simulink subsystem "Vision_Corrections_sub"  (R2023b)
settings: Solver=VariableStepAuto  StartTime=0.0  StopTime=10.0  RelTol=1e-3
undefined symbols (not defined in the file): Vision_Object_Angle_Offset, Vision_Object_X_Offset, Vision_Object_Y_Offset, Vision_Tag_Angle_Offset, Vision_Tag_X_Offset, Vision_Tag_Y_Offset
libraries: simulink_extras x2
settings Model: Creator=ander  LastModifiedBy=ander

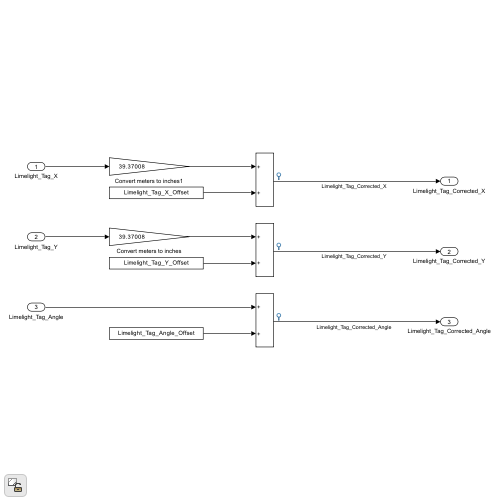
[thumbnail: Simulink's stored preview of the top-level diagram]
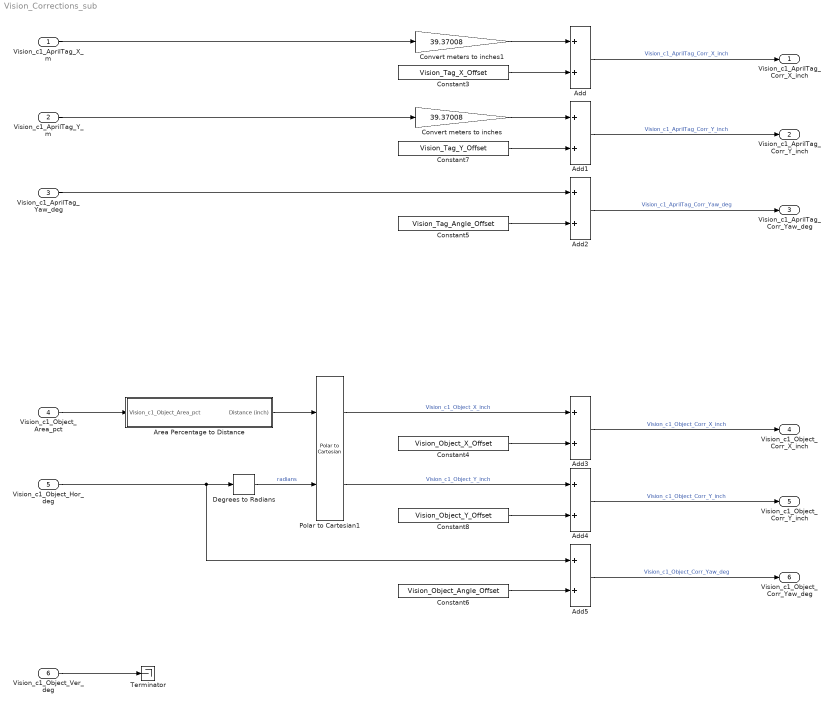
== system Vision_Corrections_sub ==
  Vision_c1_AprilTag_X_m : Inport
  Vision_c1_AprilTag_Y_m : Inport  Port=2
  Vision_c1_AprilTag_Yaw_deg : Inport  Port=3
  Vision_c1_Object_Area_pct : Inport  Port=4
  Vision_c1_Object_Hor_deg : Inport  Port=5
  Vision_c1_Object_Ver_deg : Inport  Port=6
  Add{,1..5} (6 alike) : Sum
  Area Percentage to Distance : Subsystem
  Constant3 : Constant  Value=Vision_Tag_X_Offset
  Constant4 : Constant  Value=Vision_Object_X_Offset
  Constant5 : Constant  Value=Vision_Tag_Angle_Offset
  Constant6 : Constant  Value=Vision_Object_Angle_Offset
  Constant7 : Constant  Value=Vision_Tag_Y_Offset
  Constant8 : Constant  Value=Vision_Object_Y_Offset
  Convert meters to inches : Gain  Gain=39.37008
  Convert meters to inches1 : Gain  Gain=39.37008
  Degrees to Radians : simulink_extras/Transformations/Degrees to Radians
  Polar to Cartesian1 : simulink_extras/Transformations/Polar to Cartesian
  Terminator : Terminator
  Vision_c1_AprilTag_Corr_X_inch : Outport
  Vision_c1_AprilTag_Corr_Y_inch : Outport  Port=2
  Vision_c1_AprilTag_Corr_Yaw_deg : Outport  Port=3
  Vision_c1_Object_Corr_X_inch : Outport  Port=4
  Vision_c1_Object_Corr_Y_inch : Outport  Port=5
  Vision_c1_Object_Corr_Yaw_deg : Outport  Port=6
  wires:
  Convert meters to inches1/1 -> Add/1
  Convert meters to inches/1 -> Add1/1
  Add2/1 -> Vision_c1_AprilTag_Corr_Yaw_deg/1  "Vision_c1_AprilTag_Corr_Yaw_deg"
  Add1/1 -> Vision_c1_AprilTag_Corr_Y_inch/1  "Vision_c1_AprilTag_Corr_Y_inch"
  Vision_c1_AprilTag_Y_m/1 -> Convert meters to inches/1
  Vision_c1_AprilTag_Yaw_deg/1 -> Add2/1
  Add/1 -> Vision_c1_AprilTag_Corr_X_inch/1  "Vision_c1_AprilTag_Corr_X_inch"
  Vision_c1_AprilTag_X_m/1 -> Convert meters to inches1/1
  Constant7/1 -> Add1/2
  Constant3/1 -> Add/2
  Constant5/1 -> Add2/2
  Degrees to Radians/1 -> Polar to Cartesian1/2  "radians"
  Vision_c1_Object_Hor_deg/1 -> Degrees to Radians/1, Add5/1
  Vision_c1_Object_Ver_deg/1 -> Terminator/1
  Constant4/1 -> Add3/2
  Constant8/1 -> Add4/2
  Constant6/1 -> Add5/2
  Polar to Cartesian1/1 -> Add3/1  "Vision_c1_Object_X_inch"
  Polar to Cartesian1/2 -> Add4/1  "Vision_c1_Object_Y_inch"
  Add3/1 -> Vision_c1_Object_Corr_X_inch/1  "Vision_c1_Object_Corr_X_inch"
  Add4/1 -> Vision_c1_Object_Corr_Y_inch/1  "Vision_c1_Object_Corr_Y_inch"
  Add5/1 -> Vision_c1_Object_Corr_Yaw_deg/1  "Vision_c1_Object_Corr_Yaw_deg"
  Vision_c1_Object_Area_pct/1 -> Area Percentage to Distance/1(Vision_c1_Object_Area_pct)
  Area Percentage to Distance/1(Distance (inch)) -> Polar to Cartesian1/1

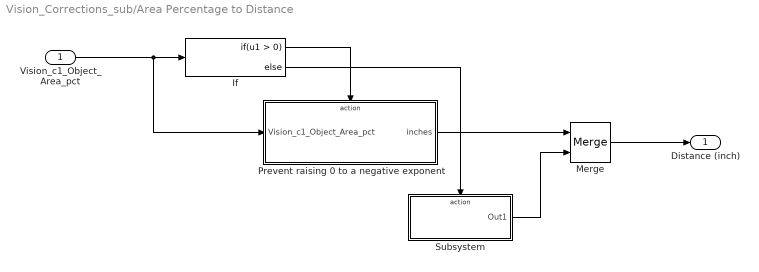
== system Vision_Corrections_sub/Area Percentage to Distance ==
  Vision_c1_Object_Area_pct : Inport
  If : If
  Merge : Merge
  Prevent raising 0 to a negative exponent : Subsystem
  Subsystem : Subsystem
  Distance (inch) : Outport
  wires:
  If/1 -> Prevent raising 0 to a negative exponent/Action
  Merge/1 -> Distance (inch)/1
  Vision_c1_Object_Area_pct/1 -> Prevent raising 0 to a negative exponent/1(Vision_c1_Object_Area_pct), If/1
  Prevent raising 0 to a negative exponent/1(inches) -> Merge/1
  If/2 -> Subsystem/Action
  Subsystem/1(Out1) -> Merge/2

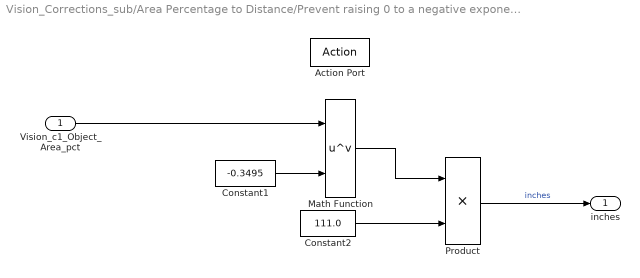
== system Vision_Corrections_sub/Area Percentage to Distance/Prevent raising 0 to a negative exponent ==
  Vision_c1_Object_Area_pct : Inport
  Action Port : ActionPort
  Constant1 : Constant  Value=-0.3495
  Constant2 : Constant  Value=111.0
  Math Function : Math  Operator=pow
  Product : Product
  inches : Outport
  wires:
  Product/1 -> inches/1  "inches"
  Vision_c1_Object_Area_pct/1 -> Math Function/1
  Constant2/1 -> Product/2
  Constant1/1 -> Math Function/2
  Math Function/1 -> Product/1

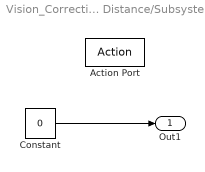
== system Vision_Corrections_sub/Area Percentage to Distance/Subsystem ==
  Action Port : ActionPort
  Constant : Constant  Value=0
  Out1 : Outport
  wires:
  Constant/1 -> Out1/1
